simulink model "vsg_stage5i_load_cycle"  (R2018b)
settings: Solver=ode23tb  StartTime=0.0  StopTime=11  MaxStep=2.5e-06  RelTol=1e-4  AbsTol=1e-6
model workspace (MAT data in the model file):
  load_increase_time_s = 3
  load_removal_time_s = 7
  secondary_Ki = 4
  secondary_Ts = 0.0001
  secondary_enable = 1
  secondary_enable_time = 0.5
  secondary_f_ref_Hz = 50
  secondary_max_pu = 0.8
  secondary_min_pu = -0.5
undefined symbols (not defined in the file): DiscIntNeverNeededParam
libraries: powerlib x40, simulink x5
settings Model: Creator=User  LastModifiedBy=User
settings DataIOCC: SaveOutput=off  SignalLogging=off  SaveTime=off  ReturnWorkspaceOutputs=on

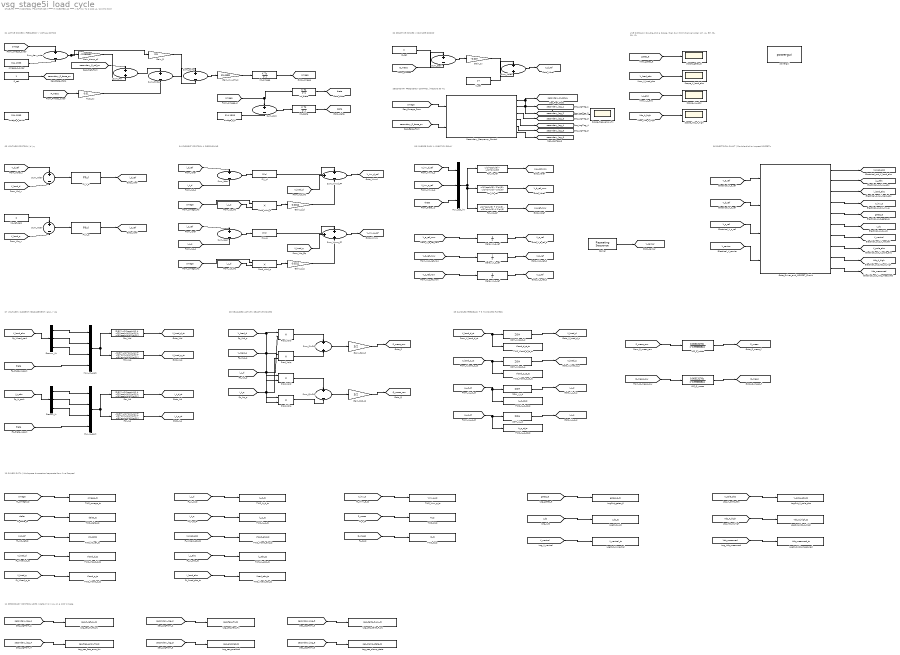
== system vsg_stage5i_load_cycle ==
  note: STAGE 5i  |  VSG CONTROL + SWITCHING MOSFET INVERTER
      | 40 V DC  /  50 Hz  /  Ts = 100 us  /  10 kHz PWM
  note: 01 ACTIVE POWER / FREQUENCY / VIRTUAL ROTOR
  note: 02 REACTIVE POWER / VOLTAGE DROOP
  note: LIVE SIGNALS  |  Double-click a Scope, then Run
      | PWM channel order: AH, AL, BH, BL, CH, CL
  note: 03 VOLTAGE CONTROL | d / q
  note: 04 CURRENT CONTROL + DECOUPLING
  note: 05 INVERSE PARK + ONE-TICK DELAY
  note: 06 ELECTRICAL PLANT | Double-click to inspect MOSFETs
  note: 07 VOLTAGE / CURRENT MEASUREMENT | abc -> dq
  note: 08 MEASURED ACTIVE / REACTIVE POWER
  note: 09 SAMPLED FEEDBACK + 5 Hz POWER FILTERS
  note: 10 SAVED DATA | Workspace timeseries (separate from live Scopes)
  note: 11 SECONDARY CONTROL LOGS | delta P is in pu on a 100 W base
  note: SECONDARY FREQUENCY CONTROL | Restore 50 Hz
  Carrier : simulink/Sources/Repeating Sequence  rep_seq_t=[0 5e-05 0.0001]  rep_seq_y=[-20 20 -20]
  Delay_V_a_ref : UnitDelay  SampleTime=0.0001
  Delay_V_b_ref : UnitDelay  SampleTime=0.0001
  Delay_V_c_ref : UnitDelay  SampleTime=0.0001
  Demux_VL : Demux  Outputs=3
  Demux_iL : Demux  Outputs=3
  Fcn_VLd : Fcn  Expr=(2/3)*( u(1)*cos(u(4)) + u(2)*cos(u(4)-2*pi/3) + u(3)*cos(u(4)+2*pi/3) )
  Fcn_VLq : Fcn  Expr=-(2/3)*( u(1)*sin(u(4)) + u(2)*sin(u(4)-2*pi/3) + u(3)*sin(u(4)+2*pi/3) )
  Fcn_Va_ref : Fcn  Expr=u(1)*cos(u(3)) - u(2)*sin(u(3))
  Fcn_Vb_ref : Fcn  Expr=u(1)*cos(u(3) - 2*pi/3) - u(2)*sin(u(3) - 2*pi/3)
  Fcn_Vc_ref : Fcn  Expr=u(1)*cos(u(3) + 2*pi/3) - u(2)*sin(u(3) + 2*pi/3)
  Fcn_iLd : Fcn  Expr=(2/3)*( u(1)*cos(u(4)) + u(2)*cos(u(4)-2*pi/3) + u(3)*cos(u(4)+2*pi/3) )
  Fcn_iLq : Fcn  Expr=-(2/3)*( u(1)*sin(u(4)) + u(2)*sin(u(4)-2*pi/3) + u(3)*sin(u(4)+2*pi/3) )
  Gain_3o2_P : Gain  Gain=3/2
  Gain_3o2_Q : Gain  Gain=3/2
  Gain_D : Gain  Gain=0.5
  Gain_Lf_d : Gain  Gain=0.0012
  Gain_Lf_q : Gain  Gain=0.0012
  Gain_droop_pf : Gain  Gain=-0.063662
  Gain_inv_2Hws : Gain  Gain=31.4159
  Gain_qv : Gain  Gain=-0.007
  Gate_Driver_and_MOSFET_Circuit : Subsystem
  Int_delta : DiscreteIntegrator  SampleTime=0.0001  ICPrevOutput=DiscIntNeverNeededParam  ICPrevScaledInput=DiscIntNeverNeededParam
  Int_omega : DiscreteIntegrator  InitialCondition=314.1593  SampleTime=0.0001  ICPrevOutput=DiscIntNeverNeededParam  ICPrevScaledInput=DiscIntNeverNeededParam
  Int_theta : DiscreteIntegrator  SampleTime=0.0001  ICPrevOutput=DiscIntNeverNeededParam  ICPrevScaledInput=DiscIntNeverNeededParam
  LPF_P_meas : DiscreteTransferFcn  Numerator=[0.00313176 0]  Denominator=[1 -0.99686824]  SampleTime=0.0001
  LPF_Q_meas : DiscreteTransferFcn  Numerator=[0.00313176 0]  Denominator=[1 -0.99686824]  SampleTime=0.0001
  LogOut_I_dc : ToWorkspace  VariableName=I_dc_ts  SaveFormat=Timeseries  SampleTime=-1
      settings: MaxDataPoints=1
  LogOut_V_neutral : ToWorkspace  VariableName=V_neutral_ts  SaveFormat=Timeseries  SampleTime=-1
      settings: MaxDataPoints=1
  LogOut_V_pole_abc : ToWorkspace  VariableName=V_pole_abc_ts  SaveFormat=Timeseries  SampleTime=-1
      settings: MaxDataPoints=1
  LogOut_Vdc_measured : ToWorkspace  VariableName=Vdc_measured_ts  SaveFormat=Timeseries  SampleTime=-1
      settings: MaxDataPoints=1
  LogOut_Vds_A_high : ToWorkspace  VariableName=Vds_A_high_ts  SaveFormat=Timeseries  SampleTime=-1
      settings: MaxDataPoints=1
  LogOut_gates_6 : ToWorkspace  VariableName=gates_6_ts  SaveFormat=Timeseries  SampleTime=-1
      settings: MaxDataPoints=1
  Log_sec_P_ref_pu : ToWorkspace  VariableName=sec_P_ref_pu_ts  SaveFormat=Timeseries
  Log_sec_clamp_state : ToWorkspace  VariableName=sec_clamp_state_ts  SaveFormat=Timeseries
  Log_sec_delta_P_pu : ToWorkspace  VariableName=sec_delta_P_pu_ts  SaveFormat=Timeseries
  Log_sec_enabled : ToWorkspace  VariableName=sec_enabled_ts  SaveFormat=Timeseries
      settings: MaxDataPoints=1
  Log_sec_freq_Hz : ToWorkspace  VariableName=sec_freq_Hz_ts  SaveFormat=Timeseries
  Log_sec_freq_error_Hz : ToWorkspace  VariableName=sec_freq_error_Hz_ts  SaveFormat=Timeseries
      settings: MaxDataPoints=1
  Mux_VL_park : Mux
  Mux_dqt_inv : Mux  Inputs=3
  Mux_iL_park : Mux
  PI_I_d : simulink/Continuous/PID Controller  Controller=PI  Form=Parallel  TimeDomain=Discrete-time  SampleTime=0.0001  IntegratorMethod=Forward Euler  FilterMethod=Forward Euler  ControllerParametersSource=internal  P=7.5396  I=314.15  D=0  UseFilter=on  N=100  TunerSelectOption=Transfer Function Based (PID Tuner App)  InitialConditionSource=internal  InitialConditionForIntegrator=0  InitialConditionForFilter=0  DifferentiatorICPrevScaledInput=0  ExternalReset=none  TrackingMode=off  Kt=1  LimitOutput=off  UpperSaturationLimit=inf  LowerSaturationLimit=-inf  LinearizeAsGain=on  AntiWindupMode=none  Kb=1  POutMin=[]  POutMax=[]  IOutMin=[]  IOutMax=[]  DOutMin=[]  DOutMax=[]  NOutMin=[]  NOutMax=[]  SumOutMin=[]  SumOutMax=[]  SaturationOutMin=[]  SaturationOutMax=[]  PParamMin=[]  PParamMax=[]  IParamMin=[]  IParamMax=[]  DParamMin=[]  DParamMax=[]  NParamMin=[]  NParamMax=[]  KbParamMin=[]  KbParamMax=[]  KtParamMin=[]  KtParamMax=[]  KbOutMin=[]  KbOutMax=[]  KtOutMin=[]  KtOutMax=[]  IntegratorOutMin=[]  IntegratorOutMax=[]  FilterOutMin=[]  FilterOutMax=[]  SumI1OutMin=[]  SumI1OutMax=[]  SumI2OutMin=[]  SumI2OutMax=[]  SumI3OutMin=[]  SumI3OutMax=[]  SumI4OutMin=[]  SumI4OutMax=[]  SumDOutMin=[]  SumDOutMax=[]  DifferentiatorOutMin=[]  DifferentiatorOutMax=[]  FilterDiffOutCoefMin=[]  FilterDiffOutCoefMax=[]  ReciprocalOutMin=[]  ReciprocalOutMax=[]  SumDenOutMin=[]  SumDenOutMax=[]  SumNumOutMin=[]  SumNumOutMax=[]  DivideOutMin=[]  DivideOutMax=[]  IntegratorContinuousStateAttributes=''  IntegratorStateMustResolveToSignalObject=off  IntegratorRTWStateStorageClass=Auto  FilterContinuousStateAttributes=''  FilterStateMustResolveToSignalObject=off  FilterRTWStateStorageClass=Auto  ParallelPVariant=InternalParameters  IdealPVariant=Disabled  IVariant=InternalParameters  DVariant=Disabled  IntegratorVariant=Discrete  SatVariant=Disabled  AWVariant=Passthrough  PCopyVariant=Disabled  TRVariant=Disabled  FdbkBlocksVariant=Forward  IdealPFdbkVariant=Disabled  SatFdbkVariant=Disabled  DerivativeFilterVariant=Disabled  NVariant=Disabled  NCopyVariant=Disabled_SignalSpec  FilterICVariant=Disabled  IntegratorICVariant=InternalICs  ExternalResetVariant=Disabled  TRSumVariant=Passthrough  SumFdbkVariant=Disabled  SumVariant=Sum_PI
  PI_I_q : simulink/Continuous/PID Controller  Controller=PI  Form=Parallel  TimeDomain=Discrete-time  SampleTime=0.0001  IntegratorMethod=Forward Euler  FilterMethod=Forward Euler  ControllerParametersSource=internal  P=7.5396  I=314.15  D=0  UseFilter=on  N=100  TunerSelectOption=Transfer Function Based (PID Tuner App)  InitialConditionSource=internal  InitialConditionForIntegrator=0  InitialConditionForFilter=0  DifferentiatorICPrevScaledInput=0  ExternalReset=none  TrackingMode=off  Kt=1  LimitOutput=off  UpperSaturationLimit=inf  LowerSaturationLimit=-inf  LinearizeAsGain=on  AntiWindupMode=none  Kb=1  POutMin=[]  POutMax=[]  IOutMin=[]  IOutMax=[]  DOutMin=[]  DOutMax=[]  NOutMin=[]  NOutMax=[]  SumOutMin=[]  SumOutMax=[]  SaturationOutMin=[]  SaturationOutMax=[]  PParamMin=[]  PParamMax=[]  IParamMin=[]  IParamMax=[]  DParamMin=[]  DParamMax=[]  NParamMin=[]  NParamMax=[]  KbParamMin=[]  KbParamMax=[]  KtParamMin=[]  KtParamMax=[]  KbOutMin=[]  KbOutMax=[]  KtOutMin=[]  KtOutMax=[]  IntegratorOutMin=[]  IntegratorOutMax=[]  FilterOutMin=[]  FilterOutMax=[]  SumI1OutMin=[]  SumI1OutMax=[]  SumI2OutMin=[]  SumI2OutMax=[]  SumI3OutMin=[]  SumI3OutMax=[]  SumI4OutMin=[]  SumI4OutMax=[]  SumDOutMin=[]  SumDOutMax=[]  DifferentiatorOutMin=[]  DifferentiatorOutMax=[]  FilterDiffOutCoefMin=[]  FilterDiffOutCoefMax=[]  ReciprocalOutMin=[]  ReciprocalOutMax=[]  SumDenOutMin=[]  SumDenOutMax=[]  SumNumOutMin=[]  SumNumOutMax=[]  DivideOutMin=[]  DivideOutMax=[]  IntegratorContinuousStateAttributes=''  IntegratorStateMustResolveToSignalObject=off  IntegratorRTWStateStorageClass=Auto  FilterContinuousStateAttributes=''  FilterStateMustResolveToSignalObject=off  FilterRTWStateStorageClass=Auto  ParallelPVariant=InternalParameters  IdealPVariant=Disabled  IVariant=InternalParameters  DVariant=Disabled  IntegratorVariant=Discrete  SatVariant=Disabled  AWVariant=Passthrough  PCopyVariant=Disabled  TRVariant=Disabled  FdbkBlocksVariant=Forward  IdealPFdbkVariant=Disabled  SatFdbkVariant=Disabled  DerivativeFilterVariant=Disabled  NVariant=Disabled  NCopyVariant=Disabled_SignalSpec  FilterICVariant=Disabled  IntegratorICVariant=InternalICs  ExternalResetVariant=Disabled  TRSumVariant=Passthrough  SumFdbkVariant=Disabled  SumVariant=Sum_PI
  PI_V_d : simulink/Continuous/PID Controller  Controller=PI  Form=Parallel  TimeDomain=Discrete-time  SampleTime=0.0001  IntegratorMethod=Forward Euler  FilterMethod=Forward Euler  ControllerParametersSource=internal  P=0.0088799  I=3.9438  D=0  UseFilter=on  N=100  TunerSelectOption=Transfer Function Based (PID Tuner App)  InitialConditionSource=internal  InitialConditionForIntegrator=0  InitialConditionForFilter=0  DifferentiatorICPrevScaledInput=0  ExternalReset=none  TrackingMode=off  Kt=1  LimitOutput=off  UpperSaturationLimit=inf  LowerSaturationLimit=-inf  LinearizeAsGain=on  AntiWindupMode=none  Kb=1  POutMin=[]  POutMax=[]  IOutMin=[]  IOutMax=[]  DOutMin=[]  DOutMax=[]  NOutMin=[]  NOutMax=[]  SumOutMin=[]  SumOutMax=[]  SaturationOutMin=[]  SaturationOutMax=[]  PParamMin=[]  PParamMax=[]  IParamMin=[]  IParamMax=[]  DParamMin=[]  DParamMax=[]  NParamMin=[]  NParamMax=[]  KbParamMin=[]  KbParamMax=[]  KtParamMin=[]  KtParamMax=[]  KbOutMin=[]  KbOutMax=[]  KtOutMin=[]  KtOutMax=[]  IntegratorOutMin=[]  IntegratorOutMax=[]  FilterOutMin=[]  FilterOutMax=[]  SumI1OutMin=[]  SumI1OutMax=[]  SumI2OutMin=[]  SumI2OutMax=[]  SumI3OutMin=[]  SumI3OutMax=[]  SumI4OutMin=[]  SumI4OutMax=[]  SumDOutMin=[]  SumDOutMax=[]  DifferentiatorOutMin=[]  DifferentiatorOutMax=[]  FilterDiffOutCoefMin=[]  FilterDiffOutCoefMax=[]  ReciprocalOutMin=[]  ReciprocalOutMax=[]  SumDenOutMin=[]  SumDenOutMax=[]  SumNumOutMin=[]  SumNumOutMax=[]  DivideOutMin=[]  DivideOutMax=[]  IntegratorContinuousStateAttributes=''  IntegratorStateMustResolveToSignalObject=off  IntegratorRTWStateStorageClass=Auto  FilterContinuousStateAttributes=''  FilterStateMustResolveToSignalObject=off  FilterRTWStateStorageClass=Auto  ParallelPVariant=InternalParameters  IdealPVariant=Disabled  IVariant=InternalParameters  DVariant=Disabled  IntegratorVariant=Discrete  SatVariant=Disabled  AWVariant=Passthrough  PCopyVariant=Disabled  TRVariant=Disabled  FdbkBlocksVariant=Forward  IdealPFdbkVariant=Disabled  SatFdbkVariant=Disabled  DerivativeFilterVariant=Disabled  NVariant=Disabled  NCopyVariant=Disabled_SignalSpec  FilterICVariant=Disabled  IntegratorICVariant=InternalICs  ExternalResetVariant=Disabled  TRSumVariant=Passthrough  SumFdbkVariant=Disabled  SumVariant=Sum_PI
  PI_V_q : simulink/Continuous/PID Controller  Controller=PI  Form=Parallel  TimeDomain=Discrete-time  SampleTime=0.0001  IntegratorMethod=Forward Euler  FilterMethod=Forward Euler  ControllerParametersSource=internal  P=0.0088799  I=3.9438  D=0  UseFilter=on  N=100  TunerSelectOption=Transfer Function Based (PID Tuner App)  InitialConditionSource=internal  InitialConditionForIntegrator=0  InitialConditionForFilter=0  DifferentiatorICPrevScaledInput=0  ExternalReset=none  TrackingMode=off  Kt=1  LimitOutput=off  UpperSaturationLimit=inf  LowerSaturationLimit=-inf  LinearizeAsGain=on  AntiWindupMode=none  Kb=1  POutMin=[]  POutMax=[]  IOutMin=[]  IOutMax=[]  DOutMin=[]  DOutMax=[]  NOutMin=[]  NOutMax=[]  SumOutMin=[]  SumOutMax=[]  SaturationOutMin=[]  SaturationOutMax=[]  PParamMin=[]  PParamMax=[]  IParamMin=[]  IParamMax=[]  DParamMin=[]  DParamMax=[]  NParamMin=[]  NParamMax=[]  KbParamMin=[]  KbParamMax=[]  KtParamMin=[]  KtParamMax=[]  KbOutMin=[]  KbOutMax=[]  KtOutMin=[]  KtOutMax=[]  IntegratorOutMin=[]  IntegratorOutMax=[]  FilterOutMin=[]  FilterOutMax=[]  SumI1OutMin=[]  SumI1OutMax=[]  SumI2OutMin=[]  SumI2OutMax=[]  SumI3OutMin=[]  SumI3OutMax=[]  SumI4OutMin=[]  SumI4OutMax=[]  SumDOutMin=[]  SumDOutMax=[]  DifferentiatorOutMin=[]  DifferentiatorOutMax=[]  FilterDiffOutCoefMin=[]  FilterDiffOutCoefMax=[]  ReciprocalOutMin=[]  ReciprocalOutMax=[]  SumDenOutMin=[]  SumDenOutMax=[]  SumNumOutMin=[]  SumNumOutMax=[]  DivideOutMin=[]  DivideOutMax=[]  IntegratorContinuousStateAttributes=''  IntegratorStateMustResolveToSignalObject=off  IntegratorRTWStateStorageClass=Auto  FilterContinuousStateAttributes=''  FilterStateMustResolveToSignalObject=off  FilterRTWStateStorageClass=Auto  ParallelPVariant=InternalParameters  IdealPVariant=Disabled  IVariant=InternalParameters  DVariant=Disabled  IntegratorVariant=Discrete  SatVariant=Disabled  AWVariant=Passthrough  PCopyVariant=Disabled  TRVariant=Disabled  FdbkBlocksVariant=Forward  IdealPFdbkVariant=Disabled  SatFdbkVariant=Disabled  DerivativeFilterVariant=Disabled  NVariant=Disabled  NCopyVariant=Disabled_SignalSpec  FilterICVariant=Disabled  IntegratorICVariant=InternalICs  ExternalResetVariant=Disabled  TRSumVariant=Passthrough  SumFdbkVariant=Disabled  SumVariant=Sum_PI
  P_set : Constant
  P_to_pu : Gain  Gain=0.01
  Prod_VdId : Product
  Prod_VdIq : Product
  Prod_VqId : Product
  Prod_VqIq : Product
  Prod_wLid_q : Product
  Prod_wLiq_d : Product
  Q_set : Constant  Value=0
  Scope_V_load_abc : Scope
  Scope_Vds_A_high : Scope
  Scope_frequency_Hz : Scope
  Scope_gates_6 : Scope
  Scope_i_L_abc : Scope
  Secondary_Frequency_Control : Subsystem
  Sum_PinDQ : Sum
  Sum_Pm : Sum
  Sum_PmPe : Sum  Inputs=+-
  Sum_Qerr : Sum  Inputs=+-
  Sum_QinDQ : Sum  Inputs=+-
  Sum_Vderr : Sum  Inputs=+-
  Sum_Vdref : Sum
  Sum_Vinvd_FF : Sum  Inputs=++-
  Sum_Vinvq_FF : Sum  Inputs=+++
  Sum_Vqerr : Sum  Inputs=+-
  Sum_dev_outer : Sum  Inputs=+-
  Sum_dom : Sum  Inputs=+-
  Sum_iderr : Sum  Inputs=+-
  Sum_iqerr : Sum  Inputs=+-
  Sum_swing : Sum  Inputs=+-
  TWS_P_ts : ToWorkspace  VariableName=P_ts  SaveFormat=Timeseries  SampleTime=-1
  TWS_Q_ts : ToWorkspace  VariableName=Q_ts  SaveFormat=Timeseries  SampleTime=-1
  TWS_Vd_ref_ts : ToWorkspace  VariableName=Vd_ref_ts  SaveFormat=Timeseries  SampleTime=-1
      settings: MaxDataPoints=1
  TWS_Vinv_a_ts : ToWorkspace  VariableName=Vinv_a_ts  SaveFormat=Timeseries  SampleTime=-1
      settings: MaxDataPoints=1
  TWS_Vload_abc_ts : ToWorkspace  VariableName=Vload_abc_ts  SaveFormat=Timeseries  SampleTime=5e-6
  TWS_Vload_d_ct_ts : ToWorkspace  VariableName=Vload_d_ct_ts  SaveFormat=Timeseries  SampleTime=-1
      settings: MaxDataPoints=1
  TWS_Vload_d_ts : ToWorkspace  VariableName=Vload_d_ts  SaveFormat=Timeseries  SampleTime=-1
      settings: MaxDataPoints=1
  TWS_Vload_q_ct_ts : ToWorkspace  VariableName=Vload_q_ct_ts  SaveFormat=Timeseries  SampleTime=-1
      settings: MaxDataPoints=1
  TWS_Vload_q_ts : ToWorkspace  VariableName=Vload_q_ts  SaveFormat=Timeseries  SampleTime=-1
      settings: MaxDataPoints=1
  TWS_delta_ts : ToWorkspace  VariableName=delta_ts  SaveFormat=Timeseries  SampleTime=-1
      settings: MaxDataPoints=1
  TWS_iL_abc_ts : ToWorkspace  VariableName=iL_abc_ts  SaveFormat=Timeseries  SampleTime=-1
      settings: MaxDataPoints=1
  TWS_iL_d_ct_ts : ToWorkspace  VariableName=iL_d_ct_ts  SaveFormat=Timeseries  SampleTime=-1
      settings: MaxDataPoints=1
  TWS_iL_d_ts : ToWorkspace  VariableName=iL_d_ts  SaveFormat=Timeseries  SampleTime=-1
      settings: MaxDataPoints=1
  TWS_iL_q_ct_ts : ToWorkspace  VariableName=iL_q_ct_ts  SaveFormat=Timeseries  SampleTime=-1
      settings: MaxDataPoints=1
  TWS_iL_q_ts : ToWorkspace  VariableName=iL_q_ts  SaveFormat=Timeseries  SampleTime=-1
      settings: MaxDataPoints=1
  TWS_iload_abc_ts : ToWorkspace  VariableName=iload_abc_ts  SaveFormat=Timeseries  SampleTime=5e-6
  TWS_omega_ts : ToWorkspace  VariableName=omega_ts  SaveFormat=Timeseries  SampleTime=-1
      settings: MaxDataPoints=1
  V_set : Constant  Value=14
  Vq_ref_zero : Constant  Value=0
  ZOH_V_load_d : ZeroOrderHold  SampleTime=0.0001
  ZOH_V_load_q : ZeroOrderHold  SampleTime=0.0001
  ZOH_i_L_d : ZeroOrderHold  SampleTime=0.0001
  ZOH_i_L_q : ZeroOrderHold  SampleTime=0.0001
  omega_s_const : Constant  Value=314.1593
  omega_s_d : Constant  Value=314.1593
  omega_s_outer : Constant  Value=314.1593
  powergui : powerlib/powergui  Priority=1  SimulationMode=Continuous  SampleTime=50e-6  frequency=50  Iterations=50  frequencyindice=60  Pbase=100e6  ErrMax=1e-4  UnitsV=kV  UnitsW=MW  buscounter=0  FunctionMessages=off  echomessages=off  EnableUseOfTLC=off  CurrentSourceSwitches=off  DisableSnubberDevices=off  DisableRonSwitches=off  DisableVfSwitches=off  DisplayEquations=off  SolverType=Tustin/Backward Euler (TBE)  Interpol=off  ExternalGateDelay=off  methode=off  Ts=100  x0status=blocks  SPID=on  SwTol=0  HookPort=off  RestoreLinks=warning  ResistiveCurrentMeasurement=off  Frange=[0:2:500]  Ylog=off  Xlog=on  ShowGrid=off  save=off  variable=ZData  structure=0  ZoomFFT=off  StartTime=0.0  cycles=1  DisplayStyle=1  fundamental=60  FreqAxis=off  MaxFrequency=1000  frequencyindicesteady=1  RmsSteady=1  display=off
  tag scope: I_dc=global, P_meas=global, P_meas_raw=global, Q_meas=global, Q_meas_raw=global, V_a_ref=global, V_a_ref_now=global, V_b_ref=global, V_b_ref_now=global, V_c_ref=global, V_c_ref_now=global, V_carrier=global, V_d_ref=global, V_inv_a=global, V_inv_d_ref=global, V_inv_q_ref=global, V_load_abc=global, V_load_d=global, V_load_d_ct=global, V_load_q=global, V_load_q_ct=global, V_neutral=global, V_pole_abc=global, Vdc_measured=global, Vds_A_high=global, delta=global, gates_6=global, i_L_abc=global, i_L_d=global, i_L_d_ct=global, i_L_q=global, i_L_q_ct=global, i_d_ref=global, i_load_abc=global, i_q_ref=global, omega=global, secondary_P_base_pu=global, secondary_P_ref_pu=global, secondary_log_1=global, secondary_log_2=global, secondary_log_3=global, secondary_log_4=global, secondary_log_5=global, secondary_log_6=global, theta=global
  wires:
  [P_meas] -> P_to_pu/1
  [omega] -> Sum_dev_outer/1
  omega_s_outer/1 -> Sum_dev_outer/2
  Sum_dev_outer/1 -> Gain_droop_pf/1, Gain_D/1
  Gain_droop_pf/1 -> Sum_Pm/2
  Sum_Pm/1 -> Sum_PmPe/1
  P_to_pu/1 -> Sum_PmPe/2
  Sum_PmPe/1 -> Sum_swing/1
  Gain_D/1 -> Sum_swing/2
  Sum_swing/1 -> Gain_inv_2Hws/1
  [omega] -> Sum_dom/1, Int_theta/1
  omega_s_d/1 -> Sum_dom/2
  [Q_meas] -> Sum_Qerr/1
  Q_set/1 -> Sum_Qerr/2
  Sum_Qerr/1 -> Gain_qv/1
  V_set/1 -> Sum_Vdref/1
  Gain_qv/1 -> Sum_Vdref/2
  Sum_Vdref/1 -> [V_d_ref]
  [V_d_ref] -> Sum_Vderr/1
  [V_load_d] -> Sum_Vderr/2
  Sum_Vderr/1 -> PI_V_d/1
  PI_V_d/1 -> [i_d_ref]
  Vq_ref_zero/1 -> Sum_Vqerr/1
  [V_load_q] -> Sum_Vqerr/2
  Sum_Vqerr/1 -> PI_V_q/1
  PI_V_q/1 -> [i_q_ref]
  [i_d_ref] -> Sum_iderr/1
  [i_L_d] -> Sum_iderr/2
  Sum_iderr/1 -> PI_I_d/1
  [omega] -> Prod_wLiq_d/1
  [i_L_q] -> Prod_wLiq_d/2
  Prod_wLiq_d/1 -> Gain_Lf_d/1
  PI_I_d/1 -> Sum_Vinvd_FF/1
  [V_load_d] -> Sum_Vinvd_FF/2
  Gain_Lf_d/1 -> Sum_Vinvd_FF/3
  Sum_Vinvd_FF/1 -> [V_inv_d_ref]
  [i_q_ref] -> Sum_iqerr/1
  [i_L_q] -> Sum_iqerr/2
  Sum_iqerr/1 -> PI_I_q/1
  [omega] -> Prod_wLid_q/1
  [i_L_d] -> Prod_wLid_q/2
  Prod_wLid_q/1 -> Gain_Lf_q/1
  PI_I_q/1 -> Sum_Vinvq_FF/1
  [V_load_q] -> Sum_Vinvq_FF/2
  Gain_Lf_q/1 -> Sum_Vinvq_FF/3
  Sum_Vinvq_FF/1 -> [V_inv_q_ref]
  [V_inv_d_ref] -> Mux_dqt_inv/1
  [V_inv_q_ref] -> Mux_dqt_inv/2
  [theta] -> Mux_dqt_inv/3
  Mux_dqt_inv/1 -> Fcn_Vb_ref/1, Fcn_Vc_ref/1, Fcn_Va_ref/1
  Fcn_Va_ref/1 -> [V_a_ref_now]
  Fcn_Vb_ref/1 -> [V_b_ref_now]
  Fcn_Vc_ref/1 -> [V_c_ref_now]
  Carrier/1 -> [V_carrier]
  [V_load_abc] -> Demux_VL/1
  Demux_VL/1 -> Mux_VL_park/1
  Demux_VL/2 -> Mux_VL_park/2
  Demux_VL/3 -> Mux_VL_park/3
  [theta] -> Mux_VL_park/4
  Mux_VL_park/1 -> Fcn_VLd/1, Fcn_VLq/1
  Fcn_VLd/1 -> [V_load_d_ct]
  Fcn_VLq/1 -> [V_load_q_ct]
  [i_L_abc] -> Demux_iL/1
  Demux_iL/1 -> Mux_iL_park/1
  Demux_iL/2 -> Mux_iL_park/2
  Demux_iL/3 -> Mux_iL_park/3
  [theta] -> Mux_iL_park/4
  Mux_iL_park/1 -> Fcn_iLd/1, Fcn_iLq/1
  Fcn_iLd/1 -> [i_L_d_ct]
  Fcn_iLq/1 -> [i_L_q_ct]
  [V_load_d] -> Prod_VdId/1, Prod_VdIq/1
  [i_L_d] -> Prod_VdId/2, Prod_VqId/2
  [V_load_q] -> Prod_VqIq/1, Prod_VqId/1
  [i_L_q] -> Prod_VqIq/2, Prod_VdIq/2
  Prod_VdId/1 -> Sum_PinDQ/1
  Prod_VqIq/1 -> Sum_PinDQ/2
  Sum_PinDQ/1 -> Gain_3o2_P/1
  Gain_3o2_P/1 -> [P_meas_raw]
  Prod_VqId/1 -> Sum_QinDQ/1
  Prod_VdIq/1 -> Sum_QinDQ/2
  Sum_QinDQ/1 -> Gain_3o2_Q/1
  Gain_3o2_Q/1 -> [Q_meas_raw]
  [omega] -> TWS_omega_ts/1
  [delta] -> TWS_delta_ts/1
  [V_d_ref] -> TWS_Vd_ref_ts/1
  [V_load_d] -> TWS_Vload_d_ts/1
  [V_load_q] -> TWS_Vload_q_ts/1
  [i_L_d] -> TWS_iL_d_ts/1
  [i_L_q] -> TWS_iL_q_ts/1
  [V_load_abc] -> TWS_Vload_abc_ts/1
  [i_L_abc] -> TWS_iL_abc_ts/1
  [i_load_abc] -> TWS_iload_abc_ts/1
  [V_inv_a] -> TWS_Vinv_a_ts/1
  [P_meas] -> TWS_P_ts/1
  [Q_meas] -> TWS_Q_ts/1
  Gain_inv_2Hws/1 -> Int_omega/1
  Int_omega/1 -> [omega]
  Int_theta/1 -> [theta]
  Sum_dom/1 -> Int_delta/1
  Int_delta/1 -> [delta]
  [V_load_d_ct] -> ZOH_V_load_d/1, TWS_Vload_d_ct_ts/1
  ZOH_V_load_d/1 -> [V_load_d]
  [V_load_q_ct] -> ZOH_V_load_q/1, TWS_Vload_q_ct_ts/1
  ZOH_V_load_q/1 -> [V_load_q]
  [i_L_d_ct] -> ZOH_i_L_d/1, TWS_iL_d_ct_ts/1
  ZOH_i_L_d/1 -> [i_L_d]
  [i_L_q_ct] -> ZOH_i_L_q/1, TWS_iL_q_ct_ts/1
  ZOH_i_L_q/1 -> [i_L_q]
  [P_meas_raw] -> LPF_P_meas/1
  LPF_P_meas/1 -> [P_meas]
  [Q_meas_raw] -> LPF_Q_meas/1
  LPF_Q_meas/1 -> [Q_meas]
  [V_a_ref_now] -> Delay_V_a_ref/1
  Delay_V_a_ref/1 -> [V_a_ref]
  [V_b_ref_now] -> Delay_V_b_ref/1
  Delay_V_b_ref/1 -> [V_b_ref]
  [V_c_ref_now] -> Delay_V_c_ref/1
  Delay_V_c_ref/1 -> [V_c_ref]
  [V_a_ref] -> Gate_Driver_and_MOSFET_Circuit/1(V_a_ref)
  [V_b_ref] -> Gate_Driver_and_MOSFET_Circuit/2(V_b_ref)
  [V_c_ref] -> Gate_Driver_and_MOSFET_Circuit/3(V_c_ref)
  [V_carrier] -> Gate_Driver_and_MOSFET_Circuit/4(V_carrier)
  Gate_Driver_and_MOSFET_Circuit/1(V_load_abc) -> [V_load_abc]
  Gate_Driver_and_MOSFET_Circuit/2(i_L_abc) -> [i_L_abc]
  Gate_Driver_and_MOSFET_Circuit/3(i_load_abc) -> [i_load_abc]
  Gate_Driver_and_MOSFET_Circuit/4(V_inv_a) -> [V_inv_a]
  Gate_Driver_and_MOSFET_Circuit/5(gates_6) -> [gates_6]
  Gate_Driver_and_MOSFET_Circuit/6(I_dc) -> [I_dc]
  Gate_Driver_and_MOSFET_Circuit/7(V_neutral) -> [V_neutral]
  Gate_Driver_and_MOSFET_Circuit/8(V_pole_abc) -> [V_pole_abc]
  Gate_Driver_and_MOSFET_Circuit/9(Vds_A_high) -> [Vds_A_high]
  Gate_Driver_and_MOSFET_Circuit/10(Vdc_measured) -> [Vdc_measured]
  [gates_6] -> Scope_gates_6/1
  [V_load_abc] -> Scope_V_load_abc/1
  [i_L_abc] -> Scope_i_L_abc/1
  [Vds_A_high] -> Scope_Vds_A_high/1
  [gates_6] -> LogOut_gates_6/1
  [I_dc] -> LogOut_I_dc/1
  [V_neutral] -> LogOut_V_neutral/1
  [V_pole_abc] -> LogOut_V_pole_abc/1
  [Vds_A_high] -> LogOut_Vds_A_high/1
  [Vdc_measured] -> LogOut_Vdc_measured/1
  P_set/1 -> [secondary_P_base_pu]
  [secondary_P_base_pu] -> Secondary_Frequency_Control/2(P_base_pu)
  [omega] -> Secondary_Frequency_Control/1(omega)
  Secondary_Frequency_Control/1(P_ref_pu) -> [secondary_P_ref_pu], [secondary_log_1]
  [secondary_P_ref_pu] -> Sum_Pm/1
  Secondary_Frequency_Control/2(f_Hz) -> Scope_frequency_Hz/1, [secondary_log_2]
  [secondary_log_1] -> Log_sec_P_ref_pu/1
  [secondary_log_2] -> Log_sec_freq_Hz/1
  Secondary_Frequency_Control/3(delta_P_pu) -> [secondary_log_3]
  [secondary_log_3] -> Log_sec_delta_P_pu/1
  Secondary_Frequency_Control/4(freq_error_Hz) -> [secondary_log_4]
  [secondary_log_4] -> Log_sec_freq_error_Hz/1
  Secondary_Frequency_Control/5(enabled) -> [secondary_log_5]
  [secondary_log_5] -> Log_sec_enabled/1
  Secondary_Frequency_Control/6(clamp_state) -> [secondary_log_6]
  [secondary_log_6] -> Log_sec_clamp_state/1

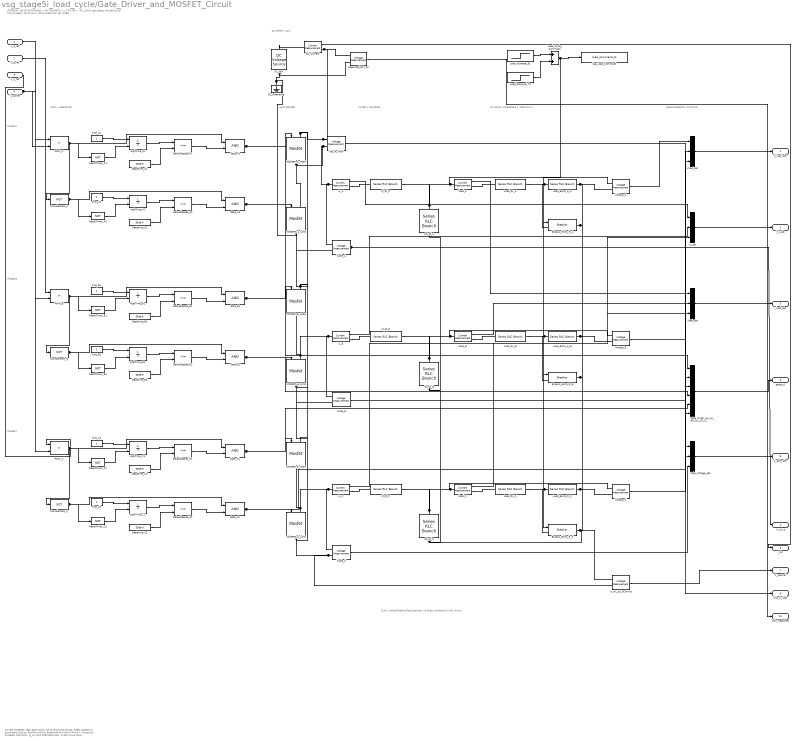
== system vsg_stage5i_load_cycle/Gate_Driver_and_MOSFET_Circuit ==
  note: Six SPS MOSFETs: logic gate inputs, not an electrical IR2104 model.
      | Deadtime assumption 520 ns; Ron=44 mOhm; diode Rd=10 mOhm/Vf=0.8 V.
      | Numerical snubbers 100 kOhm. N_AC joins filter/load stars; no DC-minus bond.
  note: STAGE 5h  |  GATE COMMANDS -> SIX MOSFETS -> LC FILTER -> RL LOAD
      | Logic gates include 520 ns turn-on delay; the driver is not an electrical Vgs model.
  note: DC SUPPLY | 40 V
  note: PWM + DEADTIME
  note: HALF BRIDGE
  note: FILTER + DAMPING
  note: RL LOAD | INCREASE 3 s / RETURN 7 s
  note: MEASUREMENTS / OUTPUTS
  note: PHASE A
  note: PHASE B
  note: PHASE C
  note: N_AC: shared floating filter/load star; no direct connection to DC minus.
  V_a_ref : Inport
  V_b_ref : Inport  Port=2
  V_c_ref : Inport  Port=3
  V_carrier : Inport  Port=4
  Bypass_Extra_R_A : powerlib/Elements/Breaker  InitialState=0  SwitchingTimes="[1/60  5/60]"  External=on  BreakerResistance=0.001  SnubberResistance=1e6  SnubberCapacitance=inf  Measurements=None  MoreParameters=on  NoBreakLoop=off
      settings: SourceProductName=Simscape Power Systems
  Bypass_Extra_R_B : powerlib/Elements/Breaker  InitialState=0  SwitchingTimes="[1/60  5/60]"  External=on  BreakerResistance=0.001  SnubberResistance=1e6  SnubberCapacitance=inf  Measurements=None  MoreParameters=on  NoBreakLoop=off
      settings: SourceProductName=Simscape Power Systems
  Bypass_Extra_R_C : powerlib/Elements/Breaker  InitialState=0  SwitchingTimes="[1/60  5/60]"  External=on  BreakerResistance=0.001  SnubberResistance=1e6  SnubberCapacitance=inf  Measurements=None  MoreParameters=on  NoBreakLoop=off
      settings: SourceProductName=Simscape Power Systems
  Complement_A : Logic  Operator=NOT  AllPortsSameDT=off  OutDataTypeStr=boolean
  Complement_B : Logic  Operator=NOT  AllPortsSameDT=off  OutDataTypeStr=boolean
  Complement_C : Logic  Operator=NOT  AllPortsSameDT=off  OutDataTypeStr=boolean
  DC_40V : powerlib/Electrical Sources/DC Voltage Source  Amplitude=40  Measurements=None
  DC_Current : powerlib/Measurements/Current Measurement  PhasorSimulation=off  OutputType=Complex  PSBequivalent=0
  DC_Reference : powerlib/Elements/Ground  LConnTagsString=a
  Deadtime_A1 : Constant  Value=520e-9
  Deadtime_A2 : Constant  Value=520e-9
  Deadtime_B1 : Constant  Value=520e-9
  Deadtime_B2 : Constant  Value=520e-9
  Deadtime_C1 : Constant  Value=520e-9
  Deadtime_C2 : Constant  Value=520e-9
  DelayElapsed_A1 : RelationalOperator  OutDataTypeStr=boolean  RndMeth=Simplest
  DelayElapsed_A2 : RelationalOperator  OutDataTypeStr=boolean  RndMeth=Simplest
  DelayElapsed_B1 : RelationalOperator  OutDataTypeStr=boolean  RndMeth=Simplest
  DelayElapsed_B2 : RelationalOperator  OutDataTypeStr=boolean  RndMeth=Simplest
  DelayElapsed_C1 : RelationalOperator  OutDataTypeStr=boolean  RndMeth=Simplest
  DelayElapsed_C2 : RelationalOperator  OutDataTypeStr=boolean  RndMeth=Simplest
  Gate_A1 : Logic  AllPortsSameDT=off  OutDataTypeStr=boolean
  Gate_A2 : Logic  AllPortsSameDT=off  OutDataTypeStr=boolean
  Gate_B1 : Logic  AllPortsSameDT=off  OutDataTypeStr=boolean
  Gate_B2 : Logic  AllPortsSameDT=off  OutDataTypeStr=boolean
  Gate_C1 : Logic  AllPortsSameDT=off  OutDataTypeStr=boolean
  Gate_C2 : Logic  AllPortsSameDT=off  OutDataTypeStr=boolean
  Gate_Order_AH_AL_BH_BL_CH_CL : Mux  Inputs=6
  HighTime_A1 : Integrator  ExternalReset=level
  HighTime_A2 : Integrator  ExternalReset=level
  HighTime_B1 : Integrator  ExternalReset=level
  HighTime_B2 : Integrator  ExternalReset=level
  HighTime_C1 : Integrator  ExternalReset=level
  HighTime_C2 : Integrator  ExternalReset=level
  Lf_Rf_A : powerlib/Elements/Series RLC Branch  LConnTagsString=__new0  RConnTagsString=__new0  BranchType=RL  Resistance=0.05  Inductance=1.2e-3  SetiL0=on  InitialCurrent=0  Capacitance=1e-6  Setx0=off  InitialVoltage=0  Measurements=None
  Lf_Rf_B : powerlib/Elements/Series RLC Branch  LConnTagsString=__new0  RConnTagsString=__new0  BranchType=RL  Resistance=0.05  Inductance=1.2e-3  SetiL0=on  InitialCurrent=0  Capacitance=1e-6  Setx0=off  InitialVoltage=0  Measurements=None
  Lf_Rf_C : powerlib/Elements/Series RLC Branch  LConnTagsString=__new0  RConnTagsString=__new0  BranchType=RL  Resistance=0.05  Inductance=1.2e-3  SetiL0=on  InitialCurrent=0  Capacitance=1e-6  Setx0=off  InitialVoltage=0  Measurements=None
  Load_Cycle_Command : Sum  SaturateOnIntegerOverflow=on  InputSameDT=on  OutDataTypeStr=Inherit: Same as first input
  Load_Extra_R_A : powerlib/Elements/Series RLC Branch  LConnTagsString=__new0  RConnTagsString=__new0  BranchType=R  Resistance=0.882  Inductance=1e-3  SetiL0=off  InitialCurrent=0  Capacitance=1e-6  Setx0=off  InitialVoltage=0  Measurements=None
  Load_Extra_R_B : powerlib/Elements/Series RLC Branch  LConnTagsString=__new0  RConnTagsString=__new0  BranchType=R  Resistance=0.882  Inductance=1e-3  SetiL0=off  InitialCurrent=0  Capacitance=1e-6  Setx0=off  InitialVoltage=0  Measurements=None
  Load_Extra_R_C : powerlib/Elements/Series RLC Branch  LConnTagsString=__new0  RConnTagsString=__new0  BranchType=R  Resistance=0.882  Inductance=1e-3  SetiL0=off  InitialCurrent=0  Capacitance=1e-6  Setx0=off  InitialVoltage=0  Measurements=None
  Load_Increase_3s : Step  Time=load_increase_time_s  SampleTime=0
  Load_RL_A : powerlib/Elements/Series RLC Branch  LConnTagsString=__new0  RConnTagsString=__new0  BranchType=RL  Resistance=2.058  Inductance=1e-3  SetiL0=on  InitialCurrent=0  Capacitance=1e-6  Setx0=off  InitialVoltage=0  Measurements=None
  Load_RL_B : powerlib/Elements/Series RLC Branch  LConnTagsString=__new0  RConnTagsString=__new0  BranchType=RL  Resistance=2.058  Inductance=1e-3  SetiL0=on  InitialCurrent=0  Capacitance=1e-6  Setx0=off  InitialVoltage=0  Measurements=None
  Load_RL_C : powerlib/Elements/Series RLC Branch  LConnTagsString=__new0  RConnTagsString=__new0  BranchType=RL  Resistance=2.058  Inductance=1e-3  SetiL0=on  InitialCurrent=0  Capacitance=1e-6  Setx0=off  InitialVoltage=0  Measurements=None
  Load_Removal_7s : Step  Time=load_removal_time_s  After=-1  SampleTime=0
  Log_Load_Command : ToWorkspace  VariableName=load_command_ts  SaveFormat=Timeseries  SampleTime=1e-4
  MOSFET_A_HIGH : powerlib/Power Electronics/Mosfet  Ron=0.044  Lon=0  Rd=0.01  Vfd=0.8  IC=0  Rs=1e5  Cs=inf  Measurements=off
  MOSFET_A_LOW : powerlib/Power Electronics/Mosfet  Ron=0.044  Lon=0  Rd=0.01  Vfd=0.8  IC=0  Rs=1e5  Cs=inf  Measurements=off
  MOSFET_B_HIGH : powerlib/Power Electronics/Mosfet  Ron=0.044  Lon=0  Rd=0.01  Vfd=0.8  IC=0  Rs=1e5  Cs=inf  Measurements=off
  MOSFET_B_LOW : powerlib/Power Electronics/Mosfet  Ron=0.044  Lon=0  Rd=0.01  Vfd=0.8  IC=0  Rs=1e5  Cs=inf  Measurements=off
  MOSFET_C_HIGH : powerlib/Power Electronics/Mosfet  Ron=0.044  Lon=0  Rd=0.01  Vfd=0.8  IC=0  Rs=1e5  Cs=inf  Measurements=off
  MOSFET_C_LOW : powerlib/Power Electronics/Mosfet  Ron=0.044  Lon=0  Rd=0.01  Vfd=0.8  IC=0  Rs=1e5  Cs=inf  Measurements=off
  Measured_DC_rail : powerlib/Measurements/Voltage Measurement  PhasorSimulation=off  OutputType=Complex  PSBequivalent=0
  N_AC_to_DCminus : powerlib/Measurements/Voltage Measurement  PhasorSimulation=off  OutputType=Complex  PSBequivalent=0
  One_A1 : Constant
  One_A2 : Constant
  One_B1 : Constant
  One_B2 : Constant
  One_C1 : Constant
  One_C2 : Constant
  PWM_A : RelationalOperator  Operator=>  OutDataTypeStr=boolean  RndMeth=Simplest
  PWM_B : RelationalOperator  Operator=>  OutDataTypeStr=boolean  RndMeth=Simplest
  PWM_C : RelationalOperator  Operator=>  OutDataTypeStr=boolean  RndMeth=Simplest
  Pole_Voltage_abc : Mux  Inputs=3
  Rd_Cf_A : powerlib/Elements/Series RLC Branch  LConnTagsString=__new0  RConnTagsString=__new0  BranchType=RC  Resistance=1  Inductance=1e-3  SetiL0=off  InitialCurrent=0  Capacitance=10e-6  Setx0=on  InitialVoltage=0  Measurements=None
  Rd_Cf_B : powerlib/Elements/Series RLC Branch  LConnTagsString=__new0  RConnTagsString=__new0  BranchType=RC  Resistance=1  Inductance=1e-3  SetiL0=off  InitialCurrent=0  Capacitance=10e-6  Setx0=on  InitialVoltage=0  Measurements=None
  Rd_Cf_C : powerlib/Elements/Series RLC Branch  LConnTagsString=__new0  RConnTagsString=__new0  BranchType=RC  Resistance=1  Inductance=1e-3  SetiL0=off  InitialCurrent=0  Capacitance=10e-6  Setx0=on  InitialVoltage=0  Measurements=None
  ResetTimer_A1 : Logic  Operator=NOT  AllPortsSameDT=off  OutDataTypeStr=boolean
  ResetTimer_A2 : Logic  Operator=NOT  AllPortsSameDT=off  OutDataTypeStr=boolean
  ResetTimer_B1 : Logic  Operator=NOT  AllPortsSameDT=off  OutDataTypeStr=boolean
  ResetTimer_B2 : Logic  Operator=NOT  AllPortsSameDT=off  OutDataTypeStr=boolean
  ResetTimer_C1 : Logic  Operator=NOT  AllPortsSameDT=off  OutDataTypeStr=boolean
  ResetTimer_C2 : Logic  Operator=NOT  AllPortsSameDT=off  OutDataTypeStr=boolean
  Vds_A_HIGH : powerlib/Measurements/Voltage Measurement  PhasorSimulation=off  OutputType=Complex  PSBequivalent=0
  Vload_abc : Mux  Inputs=3
  Vphase_A : powerlib/Measurements/Voltage Measurement  PhasorSimulation=off  OutputType=Complex  PSBequivalent=0
  Vphase_B : powerlib/Measurements/Voltage Measurement  PhasorSimulation=off  OutputType=Complex  PSBequivalent=0
  Vphase_C : powerlib/Measurements/Voltage Measurement  PhasorSimulation=off  OutputType=Complex  PSBequivalent=0
  Vpole_A : powerlib/Measurements/Voltage Measurement  PhasorSimulation=off  OutputType=Complex  PSBequivalent=0
  Vpole_B : powerlib/Measurements/Voltage Measurement  PhasorSimulation=off  OutputType=Complex  PSBequivalent=0
  Vpole_C : powerlib/Measurements/Voltage Measurement  PhasorSimulation=off  OutputType=Complex  PSBequivalent=0
  iL_A : powerlib/Measurements/Current Measurement  PhasorSimulation=off  OutputType=Complex  PSBequivalent=0
  iL_B : powerlib/Measurements/Current Measurement  PhasorSimulation=off  OutputType=Complex  PSBequivalent=0
  iL_C : powerlib/Measurements/Current Measurement  PhasorSimulation=off  OutputType=Complex  PSBequivalent=0
  iL_abc : Mux  Inputs=3
  iload_A : powerlib/Measurements/Current Measurement  PhasorSimulation=off  OutputType=Complex  PSBequivalent=0
  iload_B : powerlib/Measurements/Current Measurement  PhasorSimulation=off  OutputType=Complex  PSBequivalent=0
  iload_C : powerlib/Measurements/Current Measurement  PhasorSimulation=off  OutputType=Complex  PSBequivalent=0
  iload_abc : Mux  Inputs=3
  V_load_abc : Outport
  i_L_abc : Outport  Port=2
  i_load_abc : Outport  Port=3
  V_inv_a : Outport  Port=4
  gates_6 : Outport  Port=5
  I_dc : Outport  Port=6
  V_neutral : Outport  Port=7
  V_pole_abc : Outport  Port=8
  Vds_A_high : Outport  Port=9
  Vdc_measured : Outport  Port=10
  wires:
  V_a_ref/1 -> PWM_A/1
  V_carrier/1 -> PWM_A/2, PWM_B/2, PWM_C/2
  PWM_A/1 -> Complement_A/1, ResetTimer_A1/1, Gate_A1/1
  One_A1/1 -> HighTime_A1/1
  ResetTimer_A1/1 -> HighTime_A1/2
  HighTime_A1/1 -> DelayElapsed_A1/1
  Deadtime_A1/1 -> DelayElapsed_A1/2
  DelayElapsed_A1/1 -> Gate_A1/2
  Gate_A1/1 -> Gate_Order_AH_AL_BH_BL_CH_CL/1, MOSFET_A_HIGH/1
  Complement_A/1 -> ResetTimer_A2/1, Gate_A2/1
  One_A2/1 -> HighTime_A2/1
  ResetTimer_A2/1 -> HighTime_A2/2
  HighTime_A2/1 -> DelayElapsed_A2/1
  Deadtime_A2/1 -> DelayElapsed_A2/2
  DelayElapsed_A2/1 -> Gate_A2/2
  Gate_A2/1 -> Gate_Order_AH_AL_BH_BL_CH_CL/2, MOSFET_A_LOW/1
  Vphase_A/1 -> Vload_abc/1
  iL_A/1 -> iL_abc/1
  iload_A/1 -> iload_abc/1
  Vpole_A/1 -> Pole_Voltage_abc/1, V_inv_a/1
  V_b_ref/1 -> PWM_B/1
  PWM_B/1 -> Complement_B/1, ResetTimer_B1/1, Gate_B1/1
  One_B1/1 -> HighTime_B1/1
  ResetTimer_B1/1 -> HighTime_B1/2
  HighTime_B1/1 -> DelayElapsed_B1/1
  Deadtime_B1/1 -> DelayElapsed_B1/2
  DelayElapsed_B1/1 -> Gate_B1/2
  Gate_B1/1 -> Gate_Order_AH_AL_BH_BL_CH_CL/3, MOSFET_B_HIGH/1
  Complement_B/1 -> ResetTimer_B2/1, Gate_B2/1
  One_B2/1 -> HighTime_B2/1
  ResetTimer_B2/1 -> HighTime_B2/2
  HighTime_B2/1 -> DelayElapsed_B2/1
  Deadtime_B2/1 -> DelayElapsed_B2/2
  DelayElapsed_B2/1 -> Gate_B2/2
  Gate_B2/1 -> Gate_Order_AH_AL_BH_BL_CH_CL/4, MOSFET_B_LOW/1
  Vphase_B/1 -> Vload_abc/2
  iL_B/1 -> iL_abc/2
  iload_B/1 -> iload_abc/2
  Vpole_B/1 -> Pole_Voltage_abc/2
  V_c_ref/1 -> PWM_C/1
  PWM_C/1 -> Complement_C/1, ResetTimer_C1/1, Gate_C1/1
  One_C1/1 -> HighTime_C1/1
  ResetTimer_C1/1 -> HighTime_C1/2
  HighTime_C1/1 -> DelayElapsed_C1/1
  Deadtime_C1/1 -> DelayElapsed_C1/2
  DelayElapsed_C1/1 -> Gate_C1/2
  Gate_C1/1 -> Gate_Order_AH_AL_BH_BL_CH_CL/5, MOSFET_C_HIGH/1
  Complement_C/1 -> ResetTimer_C2/1, Gate_C2/1
  One_C2/1 -> HighTime_C2/1
  ResetTimer_C2/1 -> HighTime_C2/2
  HighTime_C2/1 -> DelayElapsed_C2/1
  Deadtime_C2/1 -> DelayElapsed_C2/2
  DelayElapsed_C2/1 -> Gate_C2/2
  Gate_C2/1 -> Gate_Order_AH_AL_BH_BL_CH_CL/6, MOSFET_C_LOW/1
  Vphase_C/1 -> Vload_abc/3
  iL_C/1 -> iL_abc/3
  iload_C/1 -> iload_abc/3
  Vpole_C/1 -> Pole_Voltage_abc/3
  Vload_abc/1 -> V_load_abc/1
  iL_abc/1 -> i_L_abc/1
  iload_abc/1 -> i_load_abc/1
  Gate_Order_AH_AL_BH_BL_CH_CL/1 -> gates_6/1
  DC_Current/1 -> I_dc/1
  N_AC_to_DCminus/1 -> V_neutral/1
  Pole_Voltage_abc/1 -> V_pole_abc/1
  Vds_A_HIGH/1 -> Vds_A_high/1
  Measured_DC_rail/1 -> Vdc_measured/1
  Load_Increase_3s/1 -> Load_Cycle_Command/1
  Load_Removal_7s/1 -> Load_Cycle_Command/2
  Load_Cycle_Command/1 -> Bypass_Extra_R_A/1, Bypass_Extra_R_B/1, Bypass_Extra_R_C/1, Log_Load_Command/1
  connections:
  DC_40V/RConn1 -- DC_Current/LConn1
  DC_40V/LConn1 -- Measured_DC_rail/LConn2 -- DC_Reference/LConn1 -- Vpole_A/LConn2 -- MOSFET_A_LOW/RConn1 -- Vpole_B/LConn2 -- MOSFET_B_LOW/RConn1 -- MOSFET_C_LOW/RConn1 -- Vpole_C/LConn2 -- N_AC_to_DCminus/LConn2
  Measured_DC_rail/LConn1 -- DC_Current/RConn1 -- Vds_A_HIGH/LConn1 -- MOSFET_A_HIGH/LConn1 -- MOSFET_B_HIGH/LConn1 -- MOSFET_C_HIGH/LConn1
  Vds_A_HIGH/LConn2 -- MOSFET_A_HIGH/RConn1 -- MOSFET_A_LOW/LConn1 -- iL_A/LConn1 -- Vpole_A/LConn1
  iL_A/RConn1 -- Lf_Rf_A/LConn1
  Rd_Cf_A/LConn1 -- Lf_Rf_A/RConn1 -- iload_A/LConn1 -- Vphase_A/LConn1
  iload_A/RConn1 -- Load_RL_A/LConn1
  Load_Extra_R_A/LConn1 -- Load_RL_A/RConn1 -- Bypass_Extra_R_A/LConn1
  MOSFET_B_LOW/LConn1 -- MOSFET_B_HIGH/RConn1 -- iL_B/LConn1 -- Vpole_B/LConn1
  iL_B/RConn1 -- Lf_Rf_B/LConn1
  Rd_Cf_B/LConn1 -- Lf_Rf_B/RConn1 -- iload_B/LConn1 -- Vphase_B/LConn1
  iload_B/RConn1 -- Load_RL_B/LConn1
  Load_Extra_R_B/LConn1 -- Load_RL_B/RConn1 -- Bypass_Extra_R_B/LConn1
  MOSFET_C_LOW/LConn1 -- MOSFET_C_HIGH/RConn1 -- iL_C/LConn1 -- Vpole_C/LConn1
  iL_C/RConn1 -- Lf_Rf_C/LConn1
  Rd_Cf_C/LConn1 -- Lf_Rf_C/RConn1 -- iload_C/LConn1 -- Vphase_C/LConn1
  iload_C/RConn1 -- Load_RL_C/LConn1
  Load_Extra_R_C/LConn1 -- Load_RL_C/RConn1 -- Bypass_Extra_R_C/LConn1
  Vphase_C/LConn2 -- Load_Extra_R_C/RConn1 -- N_AC_to_DCminus/LConn1 -- Bypass_Extra_R_C/RConn1 -- Rd_Cf_C/RConn1 -- Rd_Cf_B/RConn1 -- Rd_Cf_A/RConn1 -- Bypass_Extra_R_B/RConn1 -- Vphase_B/LConn2 -- Load_Extra_R_B/RConn1 -- Bypass_Extra_R_A/RConn1 -- Load_Extra_R_A/RConn1 -- Vphase_A/LConn2

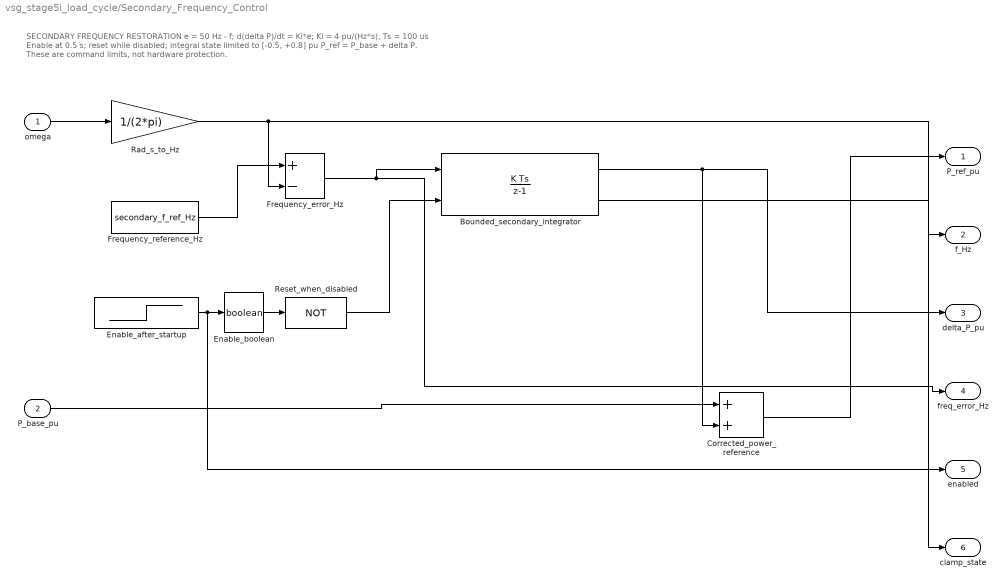
== system vsg_stage5i_load_cycle/Secondary_Frequency_Control ==
  note: SECONDARY FREQUENCY RESTORATION
      | e = 50 Hz - f; d(delta P)/dt = Ki*e; Ki = 4 pu/(Hz*s), Ts = 100 us
      | Enable at 0.5 s; reset while disabled; integral state limited to [-0.5, +0.8] pu
      | P_ref = P_base + delta P. These are command limits, not hardware protection.
  omega : Inport
  P_base_pu : Inport  Port=2
  Bounded_secondary_integrator : DiscreteIntegrator  gainval=secondary_Ki  ExternalReset=level  SampleTime=secondary_Ts  LimitOutput=on  UpperSaturationLimit=secondary_max_pu  LowerSaturationLimit=secondary_min_pu  ShowSaturationPort=on  ICPrevOutput=DiscIntNeverNeededParam  ICPrevScaledInput=DiscIntNeverNeededParam
  Corrected_power_reference : Sum  SaturateOnIntegerOverflow=on  InputSameDT=on  OutDataTypeStr=Inherit: Same as first input
  Enable_after_startup : Step  Time=secondary_enable_time  After=secondary_enable  SampleTime=secondary_Ts
  Enable_boolean : DataTypeConversion  OutDataTypeStr=boolean  SaturateOnIntegerOverflow=on  RndMeth=Zero
  Frequency_error_Hz : Sum  Inputs=+-  SaturateOnIntegerOverflow=on  InputSameDT=on  OutDataTypeStr=Inherit: Same as first input
  Frequency_reference_Hz : Constant  Value=secondary_f_ref_Hz
  Rad_s_to_Hz : Gain  Gain=1/(2*pi)  SaturateOnIntegerOverflow=on  OutDataTypeStr=Inherit: Same as input  ParamDataTypeStr=Inherit: Same as input
  Reset_when_disabled : Logic  Operator=NOT
  P_ref_pu : Outport
  f_Hz : Outport  Port=2
  delta_P_pu : Outport  Port=3
  freq_error_Hz : Outport  Port=4
  enabled : Outport  Port=5
  clamp_state : Outport  Port=6
  wires:
  omega/1 -> Rad_s_to_Hz/1
  Frequency_reference_Hz/1 -> Frequency_error_Hz/1
  Rad_s_to_Hz/1 -> Frequency_error_Hz/2, f_Hz/1
  Enable_after_startup/1 -> Enable_boolean/1, enabled/1
  Enable_boolean/1 -> Reset_when_disabled/1
  Frequency_error_Hz/1 -> Bounded_secondary_integrator/1, freq_error_Hz/1
  Reset_when_disabled/1 -> Bounded_secondary_integrator/2
  P_base_pu/1 -> Corrected_power_reference/1
  Bounded_secondary_integrator/1 -> Corrected_power_reference/2, delta_P_pu/1
  Corrected_power_reference/1 -> P_ref_pu/1
  Bounded_secondary_integrator/2 -> clamp_state/1
